simulink model "Q1"  (R2023b)
settings: Solver=FixedStepAuto  StartTime=0.0  StopTime=2000  FixedStep=0.1  RelTol=1e-3
settings Model: Creator=Arshia  LastModifiedBy=Arshia

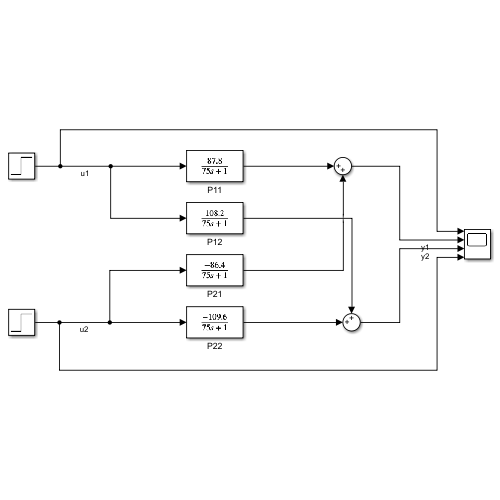
[thumbnail: Simulink's stored preview of the top-level diagram]
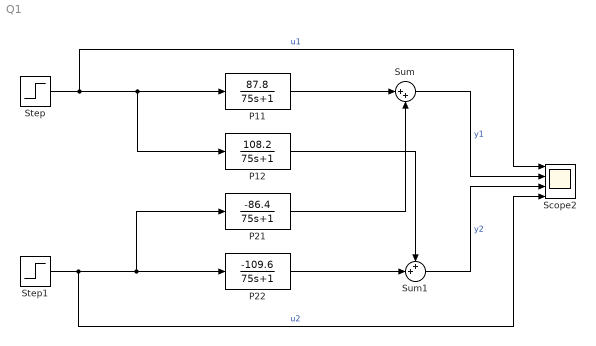
== system Q1 ==
  P11 : TransferFcn  Numerator=[87.8]  Denominator=[75 1]
  P12 : TransferFcn  Numerator=[108.2]  Denominator=[75 1]
  P21 : TransferFcn  Numerator=[-86.4]  Denominator=[75 1]
  P22 : TransferFcn  Numerator=[-109.6]  Denominator=[75 1]
  Scope2 : Scope  NumInputPorts=4
  Step : Step  Time=0  SampleTime=0
  Step1 : Step  Time=0  SampleTime=0
  Sum : Sum  Inputs=|++
  Sum1 : Sum  Inputs=++|
  wires:
  Step1/1 -> Scope2/4, P21/1, P22/1  "u2"
  Step/1 -> Scope2/1, P12/1, P11/1  "u1"
  P11/1 -> Sum/1
  P21/1 -> Sum/2
  P12/1 -> Sum1/1
  P22/1 -> Sum1/2
  Sum/1 -> Scope2/2  "y1"
  Sum1/1 -> Scope2/3  "y2"
